simulink model "generic_src"  (Simulink 10.3)
settings: Solver=ode45  StartTime=0.0  StopTime=inf  RelTol=1e-3  EnableMultiTasking=on
undefined symbols (not defined in the file or in its folder): Area_Front, Area_Rear, ay_max_off, ay_max_on, ay_per_mu_max_off, ay_per_mu_max_on, Brake_ratio, brake_valve_ctrl_kP, cat1mode1_higher, cat1mode1_lower, cat1mode2_higher, cat1mode2_lower, cat1mode3_higher, cat1mode3_lower, cat2mode1_higher, cat2mode1_lower, cat2mode2_higher, cat2mode2_lower, cat2mode3_higher, cat2mode3_lower, delta_vel, diff_lock_fac, diff_lock_off, diff_lock_on, ESP_ctrl_kD, ESP_ctrl_kI, ESP_ctrl_kP, ESP_ctrl_restore_kI, ESP_min_throttle_fac, f_ax, f_slip, g, higherlimit_highvel, higherlimit_lowvel, highervel_fac, highervelocity_fac, InitialConditionForIntegrator, limit_acc, limit_selectlow, limit_starting, limit_vdiff, locktime_throttle, lowerlimit_highvel, lowerlimit_lowvel, lowervel_fac, lowervelocity_fac, min_throttle, MPS2KMPH, MSR_ctrl_kD, MSR_ctrl_kI, MSR_ctrl_kP, MSR_min_throttle_fac, PID_kP_sideslip, PID_kP_yawrate, RADpS2RpM, rBrake, RpM2RADpS, SH_SL_switch, sideslip_vel_corr, sidesplip_deviation_max ... (+35)
libraries: CarMaker4SL x136, simulink x55, simulink_extras x6
(part 2 of 9)

== system generic_src/CarMaker/IPG Vehicle/Brake/HydBrakeCU Example/CreateBus HydBrakeCU ==
  In : Inport
  BusCreator : BusCreator  Inputs=40
  Demux : Demux  Outputs=40
      settings: DisplayOption=none
  Ground{,1..5,7..12} (12 alike) : Ground
  Terminator{1..11,15} (12 alike) : Terminator
  Out : Outport  VectorParamsAs1DForOutWhenUnconnected=off
  wires:
  In/1 -> Demux/1
  BusCreator/1 -> Out/1
  Demux/1 -> BusCreator/1  "HydBrakeCU_Out Pedal"
  Demux/2 -> BusCreator/2  "HydBrakeCU_Out Park"
  Demux/3 -> BusCreator/3  "HydBrakeCU_Out Trq_BrakeReg_trg_FL"
  Demux/4 -> BusCreator/4  "HydBrakeCU_Out Trq_BrakeReg_trg_FR"
  Demux/5 -> BusCreator/5  "HydBrakeCU_Out Trq_BrakeReg_trg_RL"
  Demux/6 -> BusCreator/6  "HydBrakeCU_Out Trq_BrakeReg_trg_RR"
  Demux/7 -> BusCreator/7  "HydBrakeCU_Out Trq_DriveSrc_trg_d0"
  Demux/8 -> BusCreator/8  "HydBrakeCU_Out Trq_DriveSrc_trg_d1"
  Demux/9 -> BusCreator/9  "HydBrakeCU_Out Trq_DriveSrc_trg_d2"
  Demux/10 -> BusCreator/10  "HydBrakeCU_Out Trq_DriveSrc_trg_d3"
  Demux/11 -> BusCreator/11  "HydBrakeCU_Out Valve_FL_Inlet"
  Demux/12 -> BusCreator/12  "HydBrakeCU_Out Valve_FR_Inlet"
  Demux/13 -> BusCreator/13  "HydBrakeCU_Out Valve_RL_Inlet"
  Demux/14 -> BusCreator/14  "HydBrakeCU_Out Valve_RR_Inlet"
  Demux/15 -> BusCreator/15  "HydBrakeCU_Out Valve_FL_Outlet"
  Demux/16 -> BusCreator/16  "HydBrakeCU_Out Valve_FR_Outlet"
  Demux/17 -> BusCreator/17  "HydBrakeCU_Out Valve_RL_Outlet"
  Demux/18 -> BusCreator/18  "HydBrakeCU_Out Valve_RR_Outlet"
  Demux/19 -> BusCreator/19  "HydBrakeCU_Out Valve_PV_1"
  Demux/20 -> BusCreator/20  "HydBrakeCU_Out Valve_PV_2"
  Demux/21 -> BusCreator/21  "HydBrakeCU_Out Valve_SV_1"
  Demux/22 -> BusCreator/22  "HydBrakeCU_Out Valve_SV_2"
  Demux/23 -> BusCreator/23  "HydBrakeCU_Out Valve_V_1"
  Demux/24 -> BusCreator/24  "HydBrakeCU_Out Valve_V_2"
  Demux/25 -> BusCreator/25  "HydBrakeCU_Out Valve_V_3"
  Demux/26 -> BusCreator/26  "HydBrakeCU_Out Valve_V_4"
  Demux/27 -> BusCreator/27  "HydBrakeCU_Out PumpCtrl"
  Demux/28 -> BusCreator/28  "HydBrakeCU_Out BooSignal"
  Demux/40 -> Terminator6/1
  Demux/39 -> Terminator7/1
  Demux/38 -> Terminator8/1
  Demux/37 -> Terminator9/1
  Demux/36 -> Terminator10/1
  Demux/35 -> Terminator11/1
  Demux/31 -> Terminator15/1
  Demux/29 -> Terminator1/1
  Ground/1 -> BusCreator/29
  Ground1/1 -> BusCreator/30
  Ground2/1 -> BusCreator/31
  Ground3/1 -> BusCreator/32
  Ground4/1 -> BusCreator/33
  Ground5/1 -> BusCreator/34
  Ground12/1 -> BusCreator/35
  Ground7/1 -> BusCreator/36
  Ground8/1 -> BusCreator/37
  Ground9/1 -> BusCreator/38
  Ground10/1 -> BusCreator/39
  Ground11/1 -> BusCreator/40
  Demux/30 -> Terminator5/1
  Demux/32 -> Terminator2/1
  Demux/33 -> Terminator3/1
  Demux/34 -> Terminator4/1

== system generic_src/CarMaker/IPG Vehicle/Brake/HydBrakeCU Example/ESP Controller ==
  note: Quantities needed by this model, but not yet available
      | at program start on CM/HIL-ds100x. Define a dummy here,
      | they will be redefined later by CarMaker.
  HydBrakeCtrl_In : Inport
  Enable : EnablePort  StatesWhenEnabling=reset
  Define CM Dict1 : CarMaker4SL/Define CM Dict  xname=PT.Engine.Trq  xunit=Nm  xmono=off  xtype=Double4  xdvaplace=None  xnstates=0  xfirststate=0  xinitial=0
  Define CM Dict11 : CarMaker4SL/Define CM Dict  xname=PT.ECU.Load_lim_max  xmono=off  xtype=Double4  xdvaplace=PTC  xnstates=0  xfirststate=0  xinitial=0
  Define CM Dict2 : CarMaker4SL/Define CM Dict  xname=PT.Gen.DL.FDiff.DVA.Trq_A2B  xunit=Nm  xmono=off  xtype=Double4  xdvaplace=VC  xnstates=0  xfirststate=0  xinitial=0
  Define CM Dict3 : CarMaker4SL/Define CM Dict  xname=PT.Clutch.0.rotv_out  xunit=rad/s  xmono=off  xtype=Double4  xdvaplace=None  xnstates=0  xfirststate=0  xinitial=0
  ESP General System : Subsystem
  ESP Input Signals : Subsystem
  Ideal Input Signals : Subsystem
  Output Signals ESP : Subsystem
  User Input Signals1 : Subsystem
  Vehicle Input Parameter : Subsystem
  HydBrakeCU_Out : Outport  VectorParamsAs1DForOutWhenUnconnected=off
  wires:
  ESP Input Signals/1(ESP Signals) -> ESP General System/1(ESP Input Signals)
  User Input Signals1/1(User_In) -> ESP General System/2(User Input Signals)
  Vehicle Input Parameter/1(Vehicle Param) -> ESP General System/3(Vehicle Input Params)
  Ideal Input Signals/1(Ideal_In) -> ESP General System/4(Ideal_In)
  Output Signals ESP/1(HydBrakeCU_Out) -> HydBrakeCU_Out/1
  HydBrakeCtrl_In/1 -> ESP Input Signals/1(HydBrakeCtrl_In)
  ESP General System/1(ESP Out) -> Output Signals ESP/1(ESP Out)

== system generic_src/CarMaker/IPG Vehicle/Brake/HydBrakeCU Example/HydBrakeCtrl_In ==
  Sync_In : Inport
  CreateBus HydBrakeCU : Subsystem
  CreateBus HydBrakeCU_Cfg : Subsystem
  CreateBus HydBrakeCtrl_In : BusCreator  Inputs=2
  S-Function : S-Function  FunctionName=cm_hydbrakectrl_in  SFunctionDeploymentMode=off  EnableBusSupport=off
  HydBrakeCtrl_In : Outport  VectorParamsAs1DForOutWhenUnconnected=off
  wires:
  Sync_In/1 -> S-Function/1
  CreateBus HydBrakeCtrl_In/1 -> HydBrakeCtrl_In/1
  S-Function/1 -> CreateBus HydBrakeCU_Cfg/1(In)
  CreateBus HydBrakeCU_Cfg/1(Out) -> CreateBus HydBrakeCtrl_In/1  "HydBrakeCU_Cfg"
  S-Function/2 -> CreateBus HydBrakeCU/1(In)
  CreateBus HydBrakeCU/1(Out) -> CreateBus HydBrakeCtrl_In/2  "HydBrakeCU"

== system generic_src/CarMaker/IPG Vehicle/Brake/HydBrakeCU Example/HydBrakeCtrl_Out ==
  HydBrakeCU : Inport
  S-Function : S-Function  FunctionName=cm_hydbrakectrl_out  SFunctionDeploymentMode=off  EnableBusSupport=off
  wires:
  HydBrakeCU/1 -> S-Function/1

== system generic_src/CarMaker/IPG Vehicle/CarAndTrailer/CarAndTrailerUpd/CreateBus Brake.IF.In ==
  In : Inport
  BusCreator : BusCreator  Inputs=9
  Demux : Demux  Outputs=9
      settings: DisplayOption=none
  Out : Outport  VectorParamsAs1DForOutWhenUnconnected=off
  wires:
  Demux/9 -> BusCreator/9  "Brake IF Trq_Reg RR"
  Demux/8 -> BusCreator/8  "Brake IF Trq_Reg RL"
  Demux/7 -> BusCreator/7  "Brake IF Trq_Reg FR"
  Demux/6 -> BusCreator/6  "Brake IF Trq_Reg FL"
  Demux/5 -> BusCreator/5  "Brake IF Trq_Reg_max RR"
  Demux/4 -> BusCreator/4  "Brake IF Trq_Reg_max RL"
  Demux/3 -> BusCreator/3  "Brake IF Trq_Reg_max FR"
  Demux/2 -> BusCreator/2  "Brake IF Trq_Reg_max FL"
  Demux/1 -> BusCreator/1  "Brake IF T_env"
  BusCreator/1 -> Out/1
  In/1 -> Demux/1

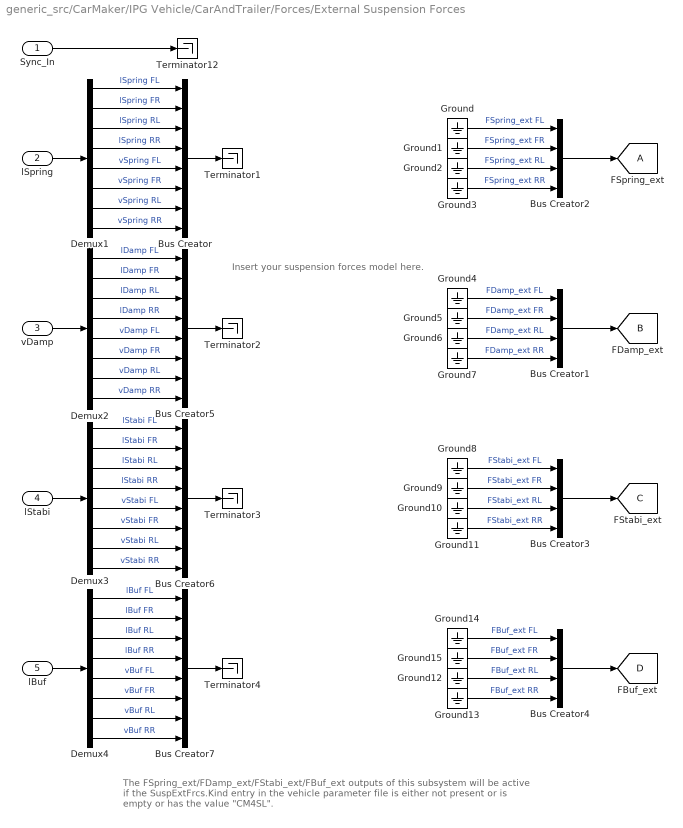
== system generic_src/CarMaker/IPG Vehicle/CarAndTrailer/Forces/External Suspension Forces ==
  note: The FSpring_ext/FDamp_ext/FStabi_ext/FBuf_ext outputs of this subsystem will be
      | active if the SuspExtFrcs.Kind entry in the vehicle parameter file
      | is either not present or is empty or has the value "CM4SL".
  note: Insert your suspension forces model here.
  Sync_In : Inport
  lSpring : Inport  Port=2
  vDamp : Inport  Port=3
  lStabi : Inport  Port=4
  lBuf : Inport  Port=5
  Bus Creator{,5..7} (4 alike) : BusCreator  Inputs=8
  Bus Creator{1..4} (4 alike) : BusCreator  Inputs=4
  Demux{1..4} (4 alike) : Demux  Outputs=8
      settings: DisplayOption=none
  Ground{,1..15} (16 alike) : Ground
  Terminator{1..4,12} (5 alike) : Terminator
  tag scope: A=global, B=global, C=global, D=global
  wires:
  Bus Creator7/1 -> Terminator4/1
  Bus Creator6/1 -> Terminator3/1
  Bus Creator5/1 -> Terminator2/1
  Bus Creator/1 -> Terminator1/1
  Demux4/8 -> Bus Creator7/8  "vBuf RR"
  Demux4/7 -> Bus Creator7/7  "vBuf RL"
  Demux4/6 -> Bus Creator7/6  "vBuf FR"
  Demux4/5 -> Bus Creator7/5  "vBuf FL"
  Demux3/8 -> Bus Creator6/8  "vStabi RR"
  Demux3/7 -> Bus Creator6/7  "vStabi RL"
  Demux3/6 -> Bus Creator6/6  "vStabi FR"
  Demux3/5 -> Bus Creator6/5  "vStabi FL"
  Demux2/8 -> Bus Creator5/8  "vDamp RR"
  Demux2/7 -> Bus Creator5/7  "vDamp RL"
  Demux2/6 -> Bus Creator5/6  "vDamp FR"
  Demux2/5 -> Bus Creator5/5  "vDamp FL"
  Demux1/8 -> Bus Creator/8  "vSpring RR"
  Demux1/7 -> Bus Creator/7  "vSpring RL"
  Demux1/6 -> Bus Creator/6  "vSpring FR"
  Demux1/5 -> Bus Creator/5  "vSpring FL"
  Demux2/4 -> Bus Creator5/4  "lDamp RR"
  Demux2/3 -> Bus Creator5/3  "lDamp RL"
  Demux2/2 -> Bus Creator5/2  "lDamp FR"
  Demux2/1 -> Bus Creator5/1  "lDamp FL"
  Demux1/4 -> Bus Creator/4  "lSpring RR"
  Demux1/3 -> Bus Creator/3  "lSpring RL"
  Demux1/2 -> Bus Creator/2  "lSpring FR"
  Demux1/1 -> Bus Creator/1  "lSpring FL"
  Demux3/4 -> Bus Creator6/4  "lStabi RR"
  Demux3/3 -> Bus Creator6/3  "lStabi RL"
  Demux3/2 -> Bus Creator6/2  "lStabi FR"
  Demux3/1 -> Bus Creator6/1  "lStabi FL"
  lStabi/1 -> Demux3/1
  vDamp/1 -> Demux2/1
  lSpring/1 -> Demux1/1
  Demux4/4 -> Bus Creator7/4  "lBuf RR"
  Demux4/3 -> Bus Creator7/3  "lBuf RL"
  Demux4/2 -> Bus Creator7/2  "lBuf FR"
  Demux4/1 -> Bus Creator7/1  "lBuf FL"
  lBuf/1 -> Demux4/1
  Ground14/1 -> Bus Creator4/1  "FBuf_ext FL"
  Ground15/1 -> Bus Creator4/2  "FBuf_ext FR"
  Ground12/1 -> Bus Creator4/3  "FBuf_ext RL"
  Ground13/1 -> Bus Creator4/4  "FBuf_ext RR"
  Bus Creator4/1 -> [D]
  Sync_In/1 -> Terminator12/1
  Bus Creator2/1 -> [A]
  Ground/1 -> Bus Creator2/1  "FSpring_ext FL"
  Ground1/1 -> Bus Creator2/2  "FSpring_ext FR"
  Ground2/1 -> Bus Creator2/3  "FSpring_ext RL"
  Ground3/1 -> Bus Creator2/4  "FSpring_ext RR"
  Ground4/1 -> Bus Creator1/1  "FDamp_ext FL"
  Ground5/1 -> Bus Creator1/2  "FDamp_ext FR"
  Ground6/1 -> Bus Creator1/3  "FDamp_ext RL"
  Ground7/1 -> Bus Creator1/4  "FDamp_ext RR"
  Bus Creator1/1 -> [B]
  Ground8/1 -> Bus Creator3/1  "FStabi_ext FL"
  Ground9/1 -> Bus Creator3/2  "FStabi_ext FR"
  Ground10/1 -> Bus Creator3/3  "FStabi_ext RL"
  Ground11/1 -> Bus Creator3/4  "FStabi_ext RR"
  Bus Creator3/1 -> [C]

== system generic_src/CarMaker/IPG Vehicle/CarAndTrailer/Forces/Suspension Forces ==
  note: <Your model here>
  note: <Your model here>
  Sync_In : Inport
  Bus Creator{,1..3,9..10} (6 alike) : BusCreator  Inputs=4
  Bus Creator{4..7} (4 alike) : BusCreator  Inputs=6
  Demux{,1..5} (6 alike) : Demux
  Demux{6..9} (4 alike) : Demux  Outputs=6
  Suspension Control Unit : S-Function  FunctionName=CM_Sfun  Parameters='ForcesSuspControl'  SFunctionDeploymentMode=off  EnableBusSupport=off
  Suspension External Forces Update : Subsystem
  Suspension Force Elements : S-Function  FunctionName=CM_Sfun  Parameters='ForcesSusp'  SFunctionDeploymentMode=off  EnableBusSupport=off
  Suspension Force Elements Update : S-Function  FunctionName=CM_Sfun  Parameters='ForcesSuspUpd'  SFunctionDeploymentMode=off  EnableBusSupport=off
  Sync_Out : Outport  VectorParamsAs1DForOutWhenUnconnected=off
  wires:
  Demux9/2 -> Bus Creator7/2  "RR DamperForce"
  Suspension Force Elements/4 -> ?
  Suspension External Forces Update/1(Out1) -> Suspension Force Elements Update/3
  Demux9/5 -> Bus Creator7/5  "RR ParasiticStiffForce"
  ? -> Suspension Force Elements Update/5
  Demux4/2 -> Bus Creator2/2  "RL DamperCtrlOut"
  Demux6/2 -> Bus Creator4/2  "FL DamperForce"
  Demux3/1 -> Bus Creator1/1  "FR SpringCtrlOut"
  Demux7/1 -> Bus Creator5/1  "FR SpringForce"
  Demux/3 -> Demux4/1  "RL"
  Demux2/1 -> Bus Creator/1  "FL SpringCtrlOut"
  Bus Creator3/1 -> Bus Creator9/4
  Demux4/1 -> Bus Creator2/1  "RL SpringCtrlOut"
  Demux/2 -> Demux3/1  "FR"
  Demux6/6 -> Bus Creator4/6  "FL ParasiticFricForce"
  Demux1/4 -> Demux9/1  "RR"
  Demux6/3 -> Bus Creator4/3  "FL StabiForce"
  Suspension Control Unit/2 -> Demux/1
  Demux3/3 -> Bus Creator1/3  "FR StabiCtrlOut"
  Demux2/4 -> Bus Creator/4  "FL BufferCtrlOut"
  Demux8/3 -> Bus Creator6/3  "RL StabiForce"
  Demux7/5 -> Bus Creator5/5  "FR ParasiticStiffForce"
  Demux6/1 -> Bus Creator4/1  "FL SpringForce"
  Suspension Force Elements/1 -> Suspension Force Elements Update/1
  Suspension Control Unit/1 -> Suspension Force Elements/1
  Demux4/4 -> Bus Creator2/4  "RL BufferCtrlOut"
  Demux3/2 -> Bus Creator1/2  "FR DamperCtrlOut"
  Demux7/4 -> Bus Creator5/4  "FR BufferForce"
  Demux9/1 -> Bus Creator7/1  "RR SpringForce"
  Bus Creator2/1 -> Bus Creator9/3
  Demux8/2 -> Bus Creator6/2  "RL DamperForce"
  ? -> Suspension Force Elements/4
  Demux1/2 -> Demux7/1  "FR"
  Demux/1 -> Demux2/1  "FL"
  Demux5/1 -> Bus Creator3/1  "RR SpringCtrlOut"
  Bus Creator1/1 -> Bus Creator9/2
  Suspension Control Unit/4 -> ?
  Sync_In/1 -> Suspension Control Unit/1
  Demux7/3 -> Bus Creator5/3  "FR StabiForce"
  Bus Creator5/1 -> Bus Creator10/2
  Demux8/6 -> Bus Creator6/6  "RL ParasiticFricForce"
  Demux9/6 -> Bus Creator7/6  "RR ParasiticFricForce"
  Suspension Force Elements/3 -> ?
  Bus Creator10/1 -> Suspension Force Elements Update/2
  ? -> Suspension Force Elements Update/4
  Demux9/4 -> Bus Creator7/4  "RR BufferForce"
  Demux7/2 -> Bus Creator5/2  "FR DamperForce"
  Demux7/6 -> Bus Creator5/6  "FR ParasiticFricForce"
  Demux2/3 -> Bus Creator/3  "FL StabiCtrlOut"
  Demux5/2 -> Bus Creator3/2  "RR DamperCtrlOut"
  Demux6/4 -> Bus Creator4/4  "FL BufferForce"
  Demux5/3 -> Bus Creator3/3  "RR StabiCtrlOut"
  Bus Creator4/1 -> Bus Creator10/1
  Suspension Force Elements/2 -> Demux1/1
  ? -> Suspension Force Elements/3
  Demux9/3 -> Bus Creator7/3  "RR StabiForce"
  Suspension Control Unit/3 -> ?
  Demux8/4 -> Bus Creator6/4  "RL BufferForce"
  Suspension Force Elements Update/1 -> Sync_Out/1
  Demux6/5 -> Bus Creator4/5  "FL ParasiticStiffForce"
  Demux5/4 -> Bus Creator3/4  "RR BufferCtrlOut"
  Demux4/3 -> Bus Creator2/3  "RL StabiCtrlOut"
  Bus Creator6/1 -> Bus Creator10/3
  Demux3/4 -> Bus Creator1/4  "FR BufferCtrlOut"
  Demux2/2 -> Bus Creator/2  "FL DamperCtrlOut"
  Bus Creator9/1 -> Suspension Force Elements/2
  Bus Creator/1 -> Bus Creator9/1
  Demux8/5 -> Bus Creator6/5  "RL ParasiticStiffForce"
  Demux1/1 -> Demux6/1  "FL"
  Demux1/3 -> Demux8/1  "RL"
  Demux8/1 -> Bus Creator6/1  "RL SpringForce"
  Demux/4 -> Demux5/1  "RR"
  Bus Creator7/1 -> Bus Creator10/4

== system generic_src/CarMaker/IPG Vehicle/CarAndTrailer/Forces/Tires ==
  note: The TireXX_Out signals will only be used if FileIdent is "CarMaker-Tire-CM4SL" in the tire parameter file!
      | An example parameter file can be found in Data/Tire/DT_CM4SL_UserTire.
  Sync_In : Inport
  TireFL_In : Inport  Port=2
  TireFR_In : Inport  Port=3
  TireRL_In : Inport  Port=4
  TireRR_In : Inport  Port=5
  Bus Creator{1..4} (4 alike) : BusCreator  Inputs=11
  Demux{1..3,8} (4 alike) : Demux  Outputs=7
      settings: DisplayOption=none
  TireFL : Subsystem
  TireFR : Subsystem
  TireRL : Subsystem
  TireRR : Subsystem
  TireFL_Out : Outport  VectorParamsAs1DForOutWhenUnconnected=off
  TireFR_Out : Outport  Port=2  VectorParamsAs1DForOutWhenUnconnected=off
  TireRL_Out : Outport  Port=3  VectorParamsAs1DForOutWhenUnconnected=off
  TireRR_Out : Outport  Port=4  VectorParamsAs1DForOutWhenUnconnected=off
  wires:
  Sync_In/1 -> TireRR/1(Sync_In), TireRL/1(Sync_In), TireFR/1(Sync_In), TireFL/1(Sync_In)
  Bus Creator4/1 -> TireRR_Out/1
  Bus Creator2/1 -> TireRL_Out/1
  Bus Creator1/1 -> TireFR_Out/1
  Demux3/5 -> TireRR/6(Rim_turnv)  "Tire_In Rim_turnv"
  Demux3/4 -> TireRR/5(Rim_rotv)  "Tire_In Rim_rotv"
  Demux3/1 -> TireRR/2(Load)  "Tire_In Load"
  Demux3/7 -> TireRR/8(muRoad)  "Tire_In mu"
  Demux3/6 -> TireRR/7(InclinAngle)  "Tire_In Camber"
  Demux3/2 -> TireRR/3(vxtrans)  "Tire_In vxtrans"
  Demux3/3 -> TireRR/4(vytrans)  "Tire_In vytrans"
  TireRR/11(AlignTrq) -> Bus Creator4/11  "Tire_Out AlignTrq"
  TireRR/10(RollResist) -> Bus Creator4/10  "Tire_Out RollResist"
  TireRR/9(OverturnTrq) -> Bus Creator4/9  "Tire_Out OverturnTrq"
  TireRR/8(LoadFrc) -> Bus Creator4/8  "Tire_Out LoadFrc"
  TireRR/7(SideFrc) -> Bus Creator4/7  "Tire_Out SideFrc"
  TireRR/6(LongFrc) -> Bus Creator4/6  "Tire_Out LongFrc"
  TireRR/5(vBelt) -> Bus Creator4/5  "Tire_Out vBelt"
  TireRR/4(rBelt_eff) -> Bus Creator4/4  "Tire_Out rBelt_eff"
  TireRR/3(TurnSlp) -> Bus Creator4/3  "Tire_Out TurnSlp"
  TireRR/1(Slp) -> Bus Creator4/1  "Tire_Out Slp"
  TireRR/2(Alpha) -> Bus Creator4/2  "Tire_Out Alpha"
  Demux2/5 -> TireRL/6(Rim_turnv)  "Tire_In Rim_turnv"
  Demux2/4 -> TireRL/5(Rim_rotv)  "Tire_In Rim_rotv"
  Demux2/1 -> TireRL/2(Load)  "Tire_In Load"
  Demux2/7 -> TireRL/8(muRoad)  "Tire_In mu"
  Demux2/6 -> TireRL/7(InclinAngle)  "Tire_In Camber"
  Demux2/2 -> TireRL/3(vxtrans)  "Tire_In vxtrans"
  Demux2/3 -> TireRL/4(vytrans)  "Tire_In vytrans"
  TireRL/11(AlignTrq) -> Bus Creator2/11  "Tire_Out AlignTrq"
  TireRL/10(RollResist) -> Bus Creator2/10  "Tire_Out RollResist"
  TireRL/9(OverturnTrq) -> Bus Creator2/9  "Tire_Out OverturnTrq"
  TireRL/8(LoadFrc) -> Bus Creator2/8  "Tire_Out LoadFrc"
  TireRL/7(SideFrc) -> Bus Creator2/7  "Tire_Out SideFrc"
  TireRL/6(LongFrc) -> Bus Creator2/6  "Tire_Out LongFrc"
  TireRL/5(vBelt) -> Bus Creator2/5  "Tire_Out vBelt"
  TireRL/4(rBelt_eff) -> Bus Creator2/4  "Tire_Out rBelt_eff"
  TireRL/3(TurnSlp) -> Bus Creator2/3  "Tire_Out TurnSlp"
  TireRL/1(Slp) -> Bus Creator2/1  "Tire_Out Slp"
  TireRL/2(Alpha) -> Bus Creator2/2  "Tire_Out Alpha"
  Demux1/5 -> TireFR/6(Rim_turnv)  "Tire_In Rim_turnv"
  Demux1/4 -> TireFR/5(Rim_rotv)  "Tire_In Rim_rotv"
  Demux1/1 -> TireFR/2(Load)  "Tire_In Load"
  Demux1/7 -> TireFR/8(muRoad)  "Tire_In mu"
  Demux1/6 -> TireFR/7(InclinAngle)  "Tire_In Camber"
  Demux1/2 -> TireFR/3(vxtrans)  "Tire_In vxtrans"
  Demux1/3 -> TireFR/4(vytrans)  "Tire_In vytrans"
  TireFR/11(AlignTrq) -> Bus Creator1/11  "Tire_Out AlignTrq"
  TireFR/10(RollResist) -> Bus Creator1/10  "Tire_Out RollResist"
  TireFR/9(OverturnTrq) -> Bus Creator1/9  "Tire_Out OverturnTrq"
  TireFR/8(LoadFrc) -> Bus Creator1/8  "Tire_Out LoadFrc"
  TireFR/7(SideFrc) -> Bus Creator1/7  "Tire_Out SideFrc"
  TireFR/6(LongFrc) -> Bus Creator1/6  "Tire_Out LongFrc"
  TireFR/5(vBelt) -> Bus Creator1/5  "Tire_Out vBelt"
  TireFR/4(rBelt_eff) -> Bus Creator1/4  "Tire_Out rBelt_eff"
  TireFR/3(TurnSlp) -> Bus Creator1/3  "Tire_Out TurnSlp"
  TireFR/1(Slp) -> Bus Creator1/1  "Tire_Out Slp"
  TireFR/2(Alpha) -> Bus Creator1/2  "Tire_Out Alpha"
  Demux8/5 -> TireFL/6(Rim_turnv)  "Tire_In Rim_turnv"
  Demux8/4 -> TireFL/5(Rim_rotv)  "Tire_In Rim_rotv"
  TireFL_In/1 -> Demux8/1
  Demux8/1 -> TireFL/2(Load)  "Tire_In Load"
  Demux8/7 -> TireFL/8(muRoad)  "Tire_In mu"
  Demux8/6 -> TireFL/7(InclinAngle)  "Tire_In Camber"
  Demux8/2 -> TireFL/3(vxtrans)  "Tire_In vxtrans"
  Demux8/3 -> TireFL/4(vytrans)  "Tire_In vytrans"
  TireFL/11(AlignTrq) -> Bus Creator3/11  "Tire_Out AlignTrq"
  TireFL/10(RollResist) -> Bus Creator3/10  "Tire_Out RollResist"
  TireFL/9(OverturnTrq) -> Bus Creator3/9  "Tire_Out OverturnTrq"
  TireFL/8(LoadFrc) -> Bus Creator3/8  "Tire_Out LoadFrc"
  TireFL/7(SideFrc) -> Bus Creator3/7  "Tire_Out SideFrc"
  TireFL/6(LongFrc) -> Bus Creator3/6  "Tire_Out LongFrc"
  TireFL/5(vBelt) -> Bus Creator3/5  "Tire_Out vBelt"
  TireFL/4(rBelt_eff) -> Bus Creator3/4  "Tire_Out rBelt_eff"
  TireFL/3(TurnSlp) -> Bus Creator3/3  "Tire_Out TurnSlp"
  TireFL/1(Slp) -> Bus Creator3/1  "Tire_Out Slp"
  TireFL/2(Alpha) -> Bus Creator3/2  "Tire_Out Alpha"
  Bus Creator3/1 -> TireFL_Out/1
  TireFR_In/1 -> Demux1/1
  TireRL_In/1 -> Demux2/1
  TireRR_In/1 -> Demux3/1

== system generic_src/CarMaker/IPG Vehicle/CarAndTrailer/Forces/Vehicle Forces ==
  Sync_In : Inport
  Bus Creator1 : BusCreator  Inputs=12
  Bus Creator8 : BusCreator  Inputs=16
  BusCreator1 : BusCreator  Inputs=4
  BusCreator2 : BusCreator  Inputs=9
  Demux : Demux  Outputs=16
      settings: DisplayOption=none
  Demux1 : Demux  Outputs=12
      settings: DisplayOption=none
  Demux2 : Demux  Outputs=13
      settings: DisplayOption=none
  Forces : S-Function  FunctionName=CM_Sfun  Parameters='Forces'  SFunctionDeploymentMode=off  EnableBusSupport=off
  Terminator : Terminator
  Sync_Out : Outport  VectorParamsAs1DForOutWhenUnconnected=off
  Car.Virtual : Outport  Port=2  VectorParamsAs1DForOutWhenUnconnected=off
  Car.Aero : Outport  Port=3  VectorParamsAs1DForOutWhenUnconnected=off
  Car.Load : Outport  Port=4  VectorParamsAs1DForOutWhenUnconnected=off
  wires:
  BusCreator1/1 -> Terminator/1  "Aero IF (in)"
  Demux2/13 -> BusCreator2/9  "car Aero Trq_1 z"
  Demux2/12 -> BusCreator2/8  "car Aero Trq_1 y"
  Demux2/11 -> BusCreator2/7  "car Aero Trq_1 x"
  Demux2/10 -> BusCreator2/6  "car Aero Frc_1 z"
  Demux2/9 -> BusCreator2/5  "car Aero Frc_1 y"
  Demux2/8 -> BusCreator2/4  "car Aero Frc_1 x"
  Demux2/7 -> BusCreator2/3  "car Aero PoA_1 z"
  Demux2/6 -> BusCreator2/2  "car Aero PoA_1 y"
  Demux2/5 -> BusCreator2/1  "car Aero PoA_1 x"
  Demux2/4 -> BusCreator1/4  "car Aero tau_1"
  Demux2/3 -> BusCreator1/3  "car Aero ApproachVel_1 z"
  Demux2/2 -> BusCreator1/2  "car Aero ApproachVel_1 y"
  Demux2/1 -> BusCreator1/1  "car Aero ApproachVel_1 x"
  Demux/16 -> Bus Creator8/16  "Car Load_3 tz"
  Demux/15 -> Bus Creator8/15  "Car Load_3 ty"
  Demux/14 -> Bus Creator8/14  "Car Load_3 tx"
  Demux/13 -> Bus Creator8/13  "Car Load_3 mass"
  Demux1/12 -> Bus Creator1/12  "Car Virtual Trq_0 z"
  Demux1/11 -> Bus Creator1/11  "Car Virtual Trq_0 y"
  Demux1/10 -> Bus Creator1/10  "Car Virtual Trq_0 x"
  Demux1/9 -> Bus Creator1/9  "Car Virtual Trq_1 z"
  Demux1/8 -> Bus Creator1/8  "Car Virtual Trq_1 y"
  Demux1/7 -> Bus Creator1/7  "Car Virtual Trq_1 x"
  Demux1/6 -> Bus Creator1/6  "Car Virtual Frc_0 z"
  Demux1/5 -> Bus Creator1/5  "Car Virtual Frc_0 y"
  Demux1/4 -> Bus Creator1/4  "Car Virtual Frc_0 x"
  Sync_In/1 -> Forces/1
  Forces/1 -> Sync_Out/1
  BusCreator2/1 -> Car.Aero/1
  Demux1/1 -> Bus Creator1/1  "Car Virtual Frc_1 x"
  Demux1/2 -> Bus Creator1/2  "Car Virtual Frc_1 y"
  Demux1/3 -> Bus Creator1/3  "Car Virtual Frc_1 z"
  Forces/3 -> Demux2/1
  Forces/2 -> Demux1/1
  Bus Creator1/1 -> Car.Virtual/1
  Bus Creator8/1 -> Car.Load/1
  Demux/1 -> Bus Creator8/1  "Car Load_0 mass"
  Demux/2 -> Bus Creator8/2  "Car Load_0 tx"
  Demux/3 -> Bus Creator8/3  "Car Load_0 ty"
  Demux/4 -> Bus Creator8/4  "Car Load_0 tz"
  Demux/5 -> Bus Creator8/5  "Car Load_1 mass"
  Demux/6 -> Bus Creator8/6  "Car Load_1 tx"
  Demux/7 -> Bus Creator8/7  "Car Load_1 ty"
  Demux/8 -> Bus Creator8/8  "Car Load_1 tz"
  Demux/9 -> Bus Creator8/9  "Car Load_2 mass"
  Demux/10 -> Bus Creator8/10  "Car Load_2 tx"
  Demux/11 -> Bus Creator8/11  "Car Load_2 ty"
  Demux/12 -> Bus Creator8/12  "Car Load_2 tz"
  Forces/4 -> Demux/1

== system generic_src/CarMaker/IPG Vehicle/CarAndTrailer/Trailer/CreateBus Car.Hitch.FrcTrq ==
  In1 : Inport
  Bus Creator7 : BusCreator  Inputs=6
  Demux7 : Demux  Outputs=6
      settings: DisplayOption=none
  Out1 : Outport  VectorParamsAs1DForOutWhenUnconnected=off
  wires:
  In1/1 -> Demux7/1
  Bus Creator7/1 -> Out1/1
  Demux7/6 -> Bus Creator7/6  "Car Hitch Trq2Car z"
  Demux7/5 -> Bus Creator7/5  "Car Hitch Trq2Car y"
  Demux7/4 -> Bus Creator7/4  "Car Hitch Trq2Car x"
  Demux7/3 -> Bus Creator7/3  "Car Hitch Frc2Car z"
  Demux7/2 -> Bus Creator7/2  "Car Hitch Frc2Car y"
  Demux7/1 -> Bus Creator7/1  "Car Hitch Frc2Car x"

== system generic_src/CarMaker/IPG Vehicle/CarAndTrailer/Trailer/CreateBus Vhcl.Motion ==
  In1 : Inport
  BusCreator : BusCreator  Inputs=15
  Demux : Demux  Outputs=15
      settings: DisplayOption=none
  Out1 : Outport  VectorParamsAs1DForOutWhenUnconnected=off
  wires:
  Demux/15 -> BusCreator/15  "Vhcl YawAcc"
  Demux/14 -> BusCreator/14  "Vhcl YawVel"
  Demux/13 -> BusCreator/13  "Vhcl Yaw"
  Demux/12 -> BusCreator/12  "Vhcl PitchAcc"
  Demux/11 -> BusCreator/11  "Vhcl PitchVel"
  Demux/10 -> BusCreator/10  "Vhcl Pitch"
  Demux/9 -> BusCreator/9  "Vhcl RollAcc"
  Demux/8 -> BusCreator/8  "Vhcl RollVel"
  Demux/7 -> BusCreator/7  "Vhcl Roll"
  Demux/6 -> BusCreator/6  "Vhcl Hitch_Pos z"
  Demux/5 -> BusCreator/5  "Vhcl Hitch_Pos y"
  Demux/4 -> BusCreator/4  "Vhcl Hitch_Pos x"
  Demux/3 -> BusCreator/3  "Vhcl sRoad"
  Demux/2 -> BusCreator/2  "Vhcl Distance"
  Demux/1 -> BusCreator/1  "Vhcl v"
  In1/1 -> Demux/1
  BusCreator/1 -> Out1/1

== system generic_src/CarMaker/IPG Vehicle/CarAndTrailer/Trailer/CreateBus Vhcl.PoI ==
  In1 : Inport
  Bus Creator3 : BusCreator  Inputs=18
  Demux3 : Demux  Outputs=18
      settings: DisplayOption=none
  Out1 : Outport  VectorParamsAs1DForOutWhenUnconnected=off
  wires:
  Demux3/18 -> Bus Creator3/18  "Vhcl PoI_GCS Elev"
  Demux3/17 -> Bus Creator3/17  "Vhcl PoI_GCS Lat"
  Demux3/16 -> Bus Creator3/16  "Vhcl PoI_GCS Long"
  Demux3/15 -> Bus Creator3/15  "Vhcl PoI_Acc_1 z"
  Demux3/14 -> Bus Creator3/14  "Vhcl PoI_Acc_1 y"
  Demux3/13 -> Bus Creator3/13  "Vhcl PoI_Acc_1 x"
  Demux3/12 -> Bus Creator3/12  "Vhcl PoI_Vel_1 z"
  Demux3/11 -> Bus Creator3/11  "Vhcl PoI_Vel_1 y"
  Demux3/10 -> Bus Creator3/10  "Vhcl PoI_Vel_1 x"
  Demux3/9 -> Bus Creator3/9  "Vhcl PoI_Acc z"
  Demux3/8 -> Bus Creator3/8  "Vhcl PoI_Acc y"
  Demux3/7 -> Bus Creator3/7  "Vhcl PoI_Acc x"
  Demux3/6 -> Bus Creator3/6  "Vhcl PoI_Vel z"
  Demux3/5 -> Bus Creator3/5  "Vhcl PoI_Vel y"
  Demux3/4 -> Bus Creator3/4  "Vhcl PoI_Vel x"
  Demux3/3 -> Bus Creator3/3  "Vhcl PoI_Pos z"
  Demux3/2 -> Bus Creator3/2  "Vhcl PoI_Pos y"
  In1/1 -> Demux3/1
  Bus Creator3/1 -> Out1/1
  Demux3/1 -> Bus Creator3/1  "Vhcl PoI_Pos x"

== system generic_src/CarMaker/IPG Vehicle/CarAndTrailer/Trailer/CreateBus Vhcl.Steering ==
  In1 : Inport
  Bus Creator3 : BusCreator  Inputs=4
  Demux : Demux
      settings: DisplayOption=none
  Out1 : Outport  VectorParamsAs1DForOutWhenUnconnected=off
  wires:
  Bus Creator3/1 -> Out1/1
  Demux/1 -> Bus Creator3/1  "Vhcl Steering Ang"
  Demux/3 -> Bus Creator3/3  "Vhcl Steering AngAcc"
  Demux/2 -> Bus Creator3/2  "Vhcl Steering AngVel"
  Demux/4 -> Bus Creator3/4  "Vhcl Steering Trq"
  In1/1 -> Demux/1

== system generic_src/CarMaker/IPG Vehicle/CarAndTrailer/Trailer/CreateBus Vhcl.Wheel.FL ==
  In1 : Inport
  Bus Creator3 : BusCreator  Inputs=14
  Demux3 : Demux  Outputs=14
      settings: DisplayOption=none
  Out1 : Outport  VectorParamsAs1DForOutWhenUnconnected=off
  wires:
  Demux3/14 -> Bus Creator3/14  "Vhcl Wheel FL Trq_WhlBearing"
  Demux3/13 -> Bus Creator3/13  "Vhcl Wheel FL Trq_T2W"
  Demux3/12 -> Bus Creator3/12  "Vhcl Wheel FL SideSlip"
  Demux3/11 -> Bus Creator3/11  "Vhcl Wheel FL LongSlip"
  Demux3/10 -> Bus Creator3/10  "Vhcl Wheel FL vBelt"
  Demux3/9 -> Bus Creator3/9  "Vhcl Wheel FL Fz"
  Demux3/8 -> Bus Creator3/8  "Vhcl Wheel FL Fy"
  Demux3/7 -> Bus Creator3/7  "Vhcl Wheel FL Fx"
  Demux3/6 -> Bus Creator3/6  "Vhcl Wheel FL r_zxy z"
  Demux3/5 -> Bus Creator3/5  "Vhcl Wheel FL r_zxy y"
  Demux3/4 -> Bus Creator3/4  "Vhcl Wheel FL r_zxy x"
  Demux3/3 -> Bus Creator3/3  "Vhcl Wheel FL t z"
  Demux3/2 -> Bus Creator3/2  "Vhcl Wheel FL t y"
  In1/1 -> Demux3/1
  Bus Creator3/1 -> Out1/1
  Demux3/1 -> Bus Creator3/1  "Vhcl Wheel FL t x"

== system generic_src/CarMaker/IPG Vehicle/CarAndTrailer/Trailer/CreateBus Vhcl.Wheel.FR ==
  In1 : Inport
  Bus Creator3 : BusCreator  Inputs=14
  Demux3 : Demux  Outputs=14
      settings: DisplayOption=none
  Out1 : Outport  VectorParamsAs1DForOutWhenUnconnected=off
  wires:
  Demux3/14 -> Bus Creator3/14  "Vhcl Wheel FR Trq_WhlBearing"
  Demux3/13 -> Bus Creator3/13  "Vhcl Wheel FR Trq_T2W"
  Demux3/12 -> Bus Creator3/12  "Vhcl Wheel FR SideSlip"
  Demux3/11 -> Bus Creator3/11  "Vhcl Wheel FR LongSlip"
  Demux3/10 -> Bus Creator3/10  "Vhcl Wheel FR vBelt"
  Demux3/9 -> Bus Creator3/9  "Vhcl Wheel FR Fz"
  Demux3/8 -> Bus Creator3/8  "Vhcl Wheel FR Fy"
  Demux3/7 -> Bus Creator3/7  "Vhcl Wheel FR Fx"
  Demux3/6 -> Bus Creator3/6  "Vhcl Wheel FR r_zxy z"
  Demux3/5 -> Bus Creator3/5  "Vhcl Wheel FR r_zxy y"
  Demux3/4 -> Bus Creator3/4  "Vhcl Wheel FR r_zxy x"
  Demux3/3 -> Bus Creator3/3  "Vhcl Wheel FR t z"
  Demux3/2 -> Bus Creator3/2  "Vhcl Wheel FR t y"
  In1/1 -> Demux3/1
  Bus Creator3/1 -> Out1/1
  Demux3/1 -> Bus Creator3/1  "Vhcl Wheel FR t x"

== system generic_src/CarMaker/IPG Vehicle/CarAndTrailer/Trailer/CreateBus Vhcl.Wheel.RL ==
  In1 : Inport
  Bus Creator3 : BusCreator  Inputs=14
  Demux3 : Demux  Outputs=14
      settings: DisplayOption=none
  Out1 : Outport  VectorParamsAs1DForOutWhenUnconnected=off
  wires:
  Demux3/14 -> Bus Creator3/14  "Vhcl Wheel RL Trq_WhlBearing"
  Demux3/13 -> Bus Creator3/13  "Vhcl Wheel RL Trq_T2W"
  Demux3/12 -> Bus Creator3/12  "Vhcl Wheel RL SideSlip"
  Demux3/11 -> Bus Creator3/11  "Vhcl Wheel RL LongSlip"
  Demux3/10 -> Bus Creator3/10  "Vhcl Wheel RL vBelt"
  Demux3/9 -> Bus Creator3/9  "Vhcl Wheel RL Fz"
  Demux3/8 -> Bus Creator3/8  "Vhcl Wheel RL Fy"
  Demux3/7 -> Bus Creator3/7  "Vhcl Wheel RL Fx"
  Demux3/6 -> Bus Creator3/6  "Vhcl Wheel RL r_zxy z"
  Demux3/5 -> Bus Creator3/5  "Vhcl Wheel RL r_zxy y"
  Demux3/4 -> Bus Creator3/4  "Vhcl Wheel RL r_zxy x"
  Demux3/3 -> Bus Creator3/3  "Vhcl Wheel RL t z"
  Demux3/2 -> Bus Creator3/2  "Vhcl Wheel RL t y"
  In1/1 -> Demux3/1
  Bus Creator3/1 -> Out1/1
  Demux3/1 -> Bus Creator3/1  "Vhcl Wheel RL t x"

== system generic_src/CarMaker/IPG Vehicle/CarAndTrailer/Trailer/CreateBus Vhcl.Wheel.RR ==
  In1 : Inport
  Bus Creator3 : BusCreator  Inputs=14
  Demux3 : Demux  Outputs=14
      settings: DisplayOption=none
  Out1 : Outport  VectorParamsAs1DForOutWhenUnconnected=off
  wires:
  Demux3/14 -> Bus Creator3/14  "Vhcl Wheel RR Trq_WhlBearing"
  Demux3/13 -> Bus Creator3/13  "Vhcl Wheel RR Trq_T2W"
  Demux3/12 -> Bus Creator3/12  "Vhcl Wheel RR SideSlip"
  Demux3/11 -> Bus Creator3/11  "Vhcl Wheel RR LongSlip"
  Demux3/10 -> Bus Creator3/10  "Vhcl Wheel RR vBelt"
  Demux3/9 -> Bus Creator3/9  "Vhcl Wheel RR Fz"
  Demux3/8 -> Bus Creator3/8  "Vhcl Wheel RR Fy"
  Demux3/7 -> Bus Creator3/7  "Vhcl Wheel RR Fx"
  Demux3/6 -> Bus Creator3/6  "Vhcl Wheel RR r_zxy z"
  Demux3/5 -> Bus Creator3/5  "Vhcl Wheel RR r_zxy y"
  Demux3/4 -> Bus Creator3/4  "Vhcl Wheel RR r_zxy x"
  Demux3/3 -> Bus Creator3/3  "Vhcl Wheel RR t z"
  Demux3/2 -> Bus Creator3/2  "Vhcl Wheel RR t y"
  In1/1 -> Demux3/1
  Bus Creator3/1 -> Out1/1
  Demux3/1 -> Bus Creator3/1  "Vhcl Wheel RR t x"

== system generic_src/CarMaker/IPG Vehicle/PowerTrain/MCU Example/CreateBus MCU ISGOut ==
  In : Inport
  BusCreator : BusCreator  Inputs=8
  Demux : Demux  Outputs=8
      settings: DisplayOption=none
  Out : Outport  VectorParamsAs1DForOutWhenUnconnected=off
  wires:
  In/1 -> Demux/1
  Demux/5 -> BusCreator/5  "MCU ISGOut Voltage_q"
  Demux/2 -> BusCreator/2  "MCU ISGOut TrqMot_max"
  Demux/1 -> BusCreator/1  "MCU ISGOut Load"
  Demux/7 -> BusCreator/7  "MCU ISGOut Voltage_v"
  Demux/8 -> BusCreator/8  "MCU ISGOut Voltage_w"
  Demux/6 -> BusCreator/6  "MCU ISGOut Voltage_u"
  Demux/4 -> BusCreator/4  "MCU ISGOut Voltage_d"
  Demux/3 -> BusCreator/3  "MCU ISGOut TrqGen_max"
  BusCreator/1 -> Out/1

== system generic_src/CarMaker/IPG Vehicle/PowerTrain/MCU Example/CreateBus MCU MotorOut0 ==
  In : Inport
  BusCreator1 : BusCreator  Inputs=8
  Demux1 : Demux  Outputs=8
      settings: DisplayOption=none
  Out : Outport  VectorParamsAs1DForOutWhenUnconnected=off
  wires:
  BusCreator1/1 -> Out/1
  Demux1/3 -> BusCreator1/3  "MCU MotorOut0 TrqGen_max"
  Demux1/2 -> BusCreator1/2  "MCU MotorOut0 TrqMot_max"
  Demux1/7 -> BusCreator1/7  "MCU MotorOut0 Voltage_v"
  Demux1/1 -> BusCreator1/1  "MCU MotorOut0 Load"
  In/1 -> Demux1/1
  Demux1/4 -> BusCreator1/4  "MCU MotorOut0 Voltage_d"
  Demux1/5 -> BusCreator1/5  "MCU MotorOut0 Voltage_q"
  Demux1/8 -> BusCreator1/8  "MCU MotorOut0 Voltage_w"
  Demux1/6 -> BusCreator1/6  "MCU MotorOut0 Voltage_u"

== system generic_src/CarMaker/IPG Vehicle/PowerTrain/MCU Example/CreateBus MCU MotorOut1 ==
  In : Inport
  BusCreator1 : BusCreator  Inputs=8
  Demux1 : Demux  Outputs=8
      settings: DisplayOption=none
  Out : Outport  VectorParamsAs1DForOutWhenUnconnected=off
  wires:
  Demux1/6 -> BusCreator1/6  "MCU MotorOut1 Voltage_u"
  Demux1/7 -> BusCreator1/7  "MCU MotorOut1 Voltage_v"
  BusCreator1/1 -> Out/1
  Demux1/3 -> BusCreator1/3  "MCU MotorOut1 TrqGen_max"
  Demux1/1 -> BusCreator1/1  "MCU MotorOut1 Load"
  In/1 -> Demux1/1
  Demux1/8 -> BusCreator1/8  "MCU MotorOut1 Voltage_w"
  Demux1/2 -> BusCreator1/2  "MCU MotorOut1 TrqMot_max"
  Demux1/4 -> BusCreator1/4  "MCU MotorOut1 Voltage_d"
  Demux1/5 -> BusCreator1/5  "MCU MotorOut1 Voltage_q"

== system generic_src/CarMaker/IPG Vehicle/PowerTrain/MCU Example/CreateBus MCU MotorOut2 ==
  In : Inport
  BusCreator1 : BusCreator  Inputs=8
  Demux1 : Demux  Outputs=8
      settings: DisplayOption=none
  Out : Outport  VectorParamsAs1DForOutWhenUnconnected=off
  wires:
  Demux1/1 -> BusCreator1/1  "MCU MotorOut2 Load"
  Demux1/3 -> BusCreator1/3  "MCU MotorOut2 TrqGen_max"
  BusCreator1/1 -> Out/1
  Demux1/8 -> BusCreator1/8  "MCU MotorOut2 Voltage_w"
  Demux1/4 -> BusCreator1/4  "MCU MotorOut2 Voltage_d"
  In/1 -> Demux1/1
  Demux1/6 -> BusCreator1/6  "MCU MotorOut2 Voltage_u"
  Demux1/2 -> BusCreator1/2  "MCU MotorOut2 TrqMot_max"
  Demux1/5 -> BusCreator1/5  "MCU MotorOut2 Voltage_q"
  Demux1/7 -> BusCreator1/7  "MCU MotorOut2 Voltage_v"

== system generic_src/CarMaker/IPG Vehicle/PowerTrain/MCU Example/CreateBus MCU MotorOut3 ==
  In : Inport
  BusCreator1 : BusCreator  Inputs=8
  Demux1 : Demux  Outputs=8
      settings: DisplayOption=none
  Out : Outport  VectorParamsAs1DForOutWhenUnconnected=off
  wires:
  Demux1/7 -> BusCreator1/7  "MCU MotorOut3 Voltage_v"
  Demux1/3 -> BusCreator1/3  "MCU MotorOut3 TrqGen_max"
  Demux1/1 -> BusCreator1/1  "MCU MotorOut3 Load"
  Demux1/5 -> BusCreator1/5  "MCU MotorOut3 Voltage_q"
  Demux1/8 -> BusCreator1/8  "MCU MotorOut3 Voltage_w"
  Demux1/4 -> BusCreator1/4  "MCU MotorOut3 Voltage_d"
  Demux1/6 -> BusCreator1/6  "MCU MotorOut3 Voltage_u"
  BusCreator1/1 -> Out/1
  In/1 -> Demux1/1
  Demux1/2 -> BusCreator1/2  "MCU MotorOut3 TrqMot_max"

== system generic_src/CarMaker/IPG Vehicle/PowerTrain/MCU Example/CreateBus MCU Status ==
  In : Inport
  BusCreator : BusCreator  Inputs=1
  Demux : Demux  Outputs=1
      settings: DisplayOption=none
  Out : Outport  VectorParamsAs1DForOutWhenUnconnected=off
  wires:
  Demux/1 -> BusCreator/1  "MCU_Out Status"
  In/1 -> Demux/1
  BusCreator/1 -> Out/1

== system generic_src/CarMaker/IPG Vehicle/PowerTrain/MCU Example/MyMotorCU ==
  Ignition : Inport
  rotv : Inport  Port=2
  Trq_trg : Inport  Port=3
  Load : Inport  Port=4
  rotv_trg : Inport  Port=5
  CfgIF : Inport  Port=6
  Bus Creator : BusCreator  Inputs=3
  Bus Selector : BusSelector  OutputSignals=MCU_Cfg ISG Ratio,TrqMot_max,TrqGen_max,MCU_Cfg ISG rotv_Mot_max,MCU_Cfg ISG rotv_Gen_max
  Bus Selector1 : BusSelector  OutputSignals=Load,TrqMot_max,TrqGen_max
  Enabled Subsystem : Subsystem  TreatAsAtomicUnit=on
  Logical Operator : Logic  Operator=NOT  AllPortsSameDT=off  OutDataTypeStr=boolean
  Merge : Merge
  ReturnZero : Subsystem  TreatAsAtomicUnit=on
  Load out : Outport  VectorParamsAs1DForOutWhenUnconnected=off
  TrqMot_max : Outport  Port=2  VectorParamsAs1DForOutWhenUnconnected=off
  TrqGen_max : Outport  Port=3  VectorParamsAs1DForOutWhenUnconnected=off
  wires:
  Bus Selector1/1 -> Load out/1  "<Load>"
  Bus Selector1/2 -> TrqMot_max/1  "<TrqMot_max>"
  Bus Selector1/3 -> TrqGen_max/1  "<TrqGen_max>"
  Merge/1 -> Bus Selector1/1
  Bus Creator/1 -> Merge/2
  ReturnZero/1(ReturnZero) -> Merge/1
  Enabled Subsystem/3(TrqGen_max) -> Bus Creator/3  "TrqGen_max"
  Enabled Subsystem/2(TrqMot_max) -> Bus Creator/2  "TrqMot_max"
  Enabled Subsystem/1(Load out) -> Bus Creator/1  "Load"
  rotv_trg/1 -> Enabled Subsystem/4(rotv_trg)
  Load/1 -> Enabled Subsystem/3(Load)
  Trq_trg/1 -> Enabled Subsystem/2(Trq_trg)
  Bus Selector/5 -> Enabled Subsystem/9(rotv_Gen_max)  "<MCU_Cfg ISG rotv_Gen_max>"
  Bus Selector/4 -> Enabled Subsystem/8(rotv_Mot_max)  "<MCU_Cfg ISG rotv_Mot_max>"
  Bus Selector/3 -> Enabled Subsystem/7(TrqGen_max table)  "<TrqGen_max>"
  Bus Selector/2 -> Enabled Subsystem/6(TrqMot_max table)  "<TrqMot_max >"
  Bus Selector/1 -> Enabled Subsystem/5(Ratio)  "<MCU_Cfg ISG Ratio>"
  CfgIF/1 -> Bus Selector/1
  rotv/1 -> Enabled Subsystem/1(rotv)
  Logical Operator/1 -> ReturnZero/Enable
  Ignition/1 -> Logical Operator/1, Enabled Subsystem/Enable

== system generic_src/CarMaker/IPG Vehicle/PowerTrain/MCU Example/PTMotorCU_In ==
  Sync_In : Inport
  CreateBus MCU ISGIn : Subsystem
  CreateBus MCU ISGOut : Subsystem
  CreateBus MCU Ignition : Subsystem
  CreateBus MCU MotorIn0 : Subsystem
  CreateBus MCU MotorIn1 : Subsystem
  CreateBus MCU MotorIn2 : Subsystem
  CreateBus MCU MotorIn3 : Subsystem
  CreateBus MCU MotorOut0 : Subsystem
  CreateBus MCU MotorOut1 : Subsystem
  CreateBus MCU MotorOut2 : Subsystem
  CreateBus MCU MotorOut3 : Subsystem
  CreateBus MCU_Cfg ISG : Subsystem
  CreateBus MCU_Cfg Misc : Subsystem
  CreateBus MCU_Cfg Motor0 : Subsystem
  CreateBus MCU_Cfg Motor1 : Subsystem
  CreateBus MCU_Cfg Motor2 : Subsystem
  CreateBus MCU_Cfg Motor3 : Subsystem
  CreateBus PTMotorCU_In : BusCreator  Inputs=17
  S-Function : S-Function  FunctionName=cm_ptmotorcu_in  SFunctionDeploymentMode=off  EnableBusSupport=off
  PTMotorCU_In : Outport  VectorParamsAs1DForOutWhenUnconnected=off
  wires:
  S-Function/17 -> CreateBus MCU MotorOut3/1(In)
  S-Function/16 -> CreateBus MCU MotorOut2/1(In)
  S-Function/15 -> CreateBus MCU MotorOut1/1(In)
  S-Function/12 -> CreateBus MCU MotorIn2/1(In)
  S-Function/10 -> CreateBus MCU MotorIn0/1(In)
  CreateBus MCU MotorIn0/1(Out) -> CreateBus PTMotorCU_In/10  "MCU MotorIn0"
  CreateBus MCU ISGIn/1(Out) -> CreateBus PTMotorCU_In/8  "MCU ISGIn"
  CreateBus MCU MotorIn2/1(Out) -> CreateBus PTMotorCU_In/12  "MCU MotorIn2"
  S-Function/8 -> CreateBus MCU ISGIn/1(In)
  CreateBus MCU_Cfg ISG/1(Out) -> CreateBus PTMotorCU_In/2  "MCU_Cfg ISG"
  CreateBus MCU MotorIn3/1(Out) -> CreateBus PTMotorCU_In/13  "MCU MotorIn3"
  CreateBus MCU MotorIn1/1(Out) -> CreateBus PTMotorCU_In/11  "MCU MotorIn1"
  S-Function/14 -> CreateBus MCU MotorOut0/1(In)
  S-Function/13 -> CreateBus MCU MotorIn3/1(In)
  S-Function/11 -> CreateBus MCU MotorIn1/1(In)
  CreateBus MCU ISGOut/1(Out) -> CreateBus PTMotorCU_In/9  "MCU ISGOut"
  CreateBus MCU_Cfg Misc/1(Out) -> CreateBus PTMotorCU_In/1  "MCU_Cfg Misc"
  CreateBus MCU Ignition/1(Out) -> CreateBus PTMotorCU_In/7  "MCU Ignition"
  S-Function/3 -> CreateBus MCU_Cfg Motor0/1(In)
  Sync_In/1 -> S-Function/1
  CreateBus MCU MotorOut2/1(Out) -> CreateBus PTMotorCU_In/16  "MCU MotorOut2"
  CreateBus MCU MotorOut0/1(Out) -> CreateBus PTMotorCU_In/14  "MCU MotorOut0"
  CreateBus MCU MotorOut1/1(Out) -> CreateBus PTMotorCU_In/15  "MCU MotorOut1"
  CreateBus MCU_Cfg Motor2/1(Out) -> CreateBus PTMotorCU_In/5  "MCU_Cfg Motor2"
  S-Function/2 -> CreateBus MCU_Cfg ISG/1(In)
  CreateBus MCU_Cfg Motor3/1(Out) -> CreateBus PTMotorCU_In/6  "MCU_Cfg Motor3"
  S-Function/5 -> CreateBus MCU_Cfg Motor2/1(In)
  CreateBus MCU_Cfg Motor1/1(Out) -> CreateBus PTMotorCU_In/4  "MCU_Cfg Motor1"
  S-Function/1 -> CreateBus MCU_Cfg Misc/1(In)
  S-Function/4 -> CreateBus MCU_Cfg Motor1/1(In)
  CreateBus MCU_Cfg Motor0/1(Out) -> CreateBus PTMotorCU_In/3  "MCU_Cfg Motor0"
  CreateBus PTMotorCU_In/1 -> PTMotorCU_In/1
  CreateBus MCU MotorOut3/1(Out) -> CreateBus PTMotorCU_In/17  "MCU MotorOut3"
  S-Function/9 -> CreateBus MCU ISGOut/1(In)
  S-Function/6 -> CreateBus MCU_Cfg Motor3/1(In)
  S-Function/7 -> CreateBus MCU Ignition/1(In)

== system generic_src/CarMaker/IPG Vehicle/PowerTrain/MCU Example/PTMotorCU_Out ==
  MCU Status : Inport
  MCU ISGOut : Inport  Port=2
  MCU MotorOut0 : Inport  Port=3
  MCU MotorOut1 : Inport  Port=4
  MCU MotorOut2 : Inport  Port=5
  MCU MotorOut3 : Inport  Port=6
  S-Function : S-Function  FunctionName=cm_ptmotorcu_out  SFunctionDeploymentMode=off  EnableBusSupport=off
  wires:
  MCU MotorOut3/1 -> S-Function/6
  MCU MotorOut1/1 -> S-Function/4
  MCU MotorOut0/1 -> S-Function/3
  MCU MotorOut2/1 -> S-Function/5
  MCU Status/1 -> S-Function/1
  MCU ISGOut/1 -> S-Function/2

== system generic_src/CarMaker/IPG Vehicle/PowerTrain/PTControl Example/CreateBus PTC BatteryHVOut ==
  In : Inport
  BusCreator : BusCreator  Inputs=2
  Demux : Demux  Outputs=2
      settings: DisplayOption=none
  Out : Outport  VectorParamsAs1DForOutWhenUnconnected=off
  wires:
  Demux/2 -> BusCreator/2  "PTC BattHVOut MassFlowCool_trg"
  Demux/1 -> BusCreator/1  "PTC BattHVOut Temp_trg"
  In/1 -> Demux/1
  BusCreator/1 -> Out/1

== system generic_src/CarMaker/IPG Vehicle/PowerTrain/PTControl Example/CreateBus PTC BatteryLVOut ==
  In : Inport
  BusCreator : BusCreator  Inputs=2
  Demux : Demux  Outputs=2
      settings: DisplayOption=none
  Out : Outport  VectorParamsAs1DForOutWhenUnconnected=off
  wires:
  Demux/2 -> BusCreator/2  "PTC BattLVOut MassFlowCool_trg"
  In/1 -> Demux/1
  Demux/1 -> BusCreator/1  "PTC BattLVOut Temp_trg"
  BusCreator/1 -> Out/1

== system generic_src/CarMaker/IPG Vehicle/PowerTrain/PTControl Example/CreateBus PTC EngineOut ==
  In : Inport
  BusCreator : BusCreator  Inputs=5
  Demux : Demux  Outputs=5
      settings: DisplayOption=none
  Out : Outport  VectorParamsAs1DForOutWhenUnconnected=off
  wires:
  Demux/5 -> BusCreator/5  "PTC EngineOut rotv_trg"
  Demux/4 -> BusCreator/4  "PTC EngineOut Trq_trg"
  Demux/3 -> BusCreator/3  "PTC EngineOut Load"
  Demux/2 -> BusCreator/2  "PTC EngineOut FuelCutOff"
  Demux/1 -> BusCreator/1  "PTC EngineOut set_ISC"
  BusCreator/1 -> Out/1
  In/1 -> Demux/1

== system generic_src/CarMaker/IPG Vehicle/PowerTrain/PTControl Example/CreateBus PTC ISGOut ==
  In : Inport
  BusCreator : BusCreator  Inputs=3
  Demux : Demux  Outputs=3
      settings: DisplayOption=none
  Out : Outport  VectorParamsAs1DForOutWhenUnconnected=off
  wires:
  Demux/3 -> BusCreator/3  "PTC ISGOut rotv_trg"
  Demux/2 -> BusCreator/2  "PTC ISGOut Trq_trg"
  Demux/1 -> BusCreator/1  "PTC ISGOut Load"
  BusCreator/1 -> Out/1
  In/1 -> Demux/1

== system generic_src/CarMaker/IPG Vehicle/PowerTrain/PTControl Example/CreateBus PTC MiscOut ==
  In : Inport
  BusCreator : BusCreator  Inputs=4
  Demux : Demux
      settings: DisplayOption=none
  Out : Outport  VectorParamsAs1DForOutWhenUnconnected=off
  wires:
  Demux/4 -> BusCreator/4  "PTC_Out Ignition"
  Demux/3 -> BusCreator/3  "PTC_Out StrategyMode"
  Demux/2 -> BusCreator/2  "PTC_Out OperationError"
  Demux/1 -> BusCreator/1  "PTC_Out OperationState"
  BusCreator/1 -> Out/1
  In/1 -> Demux/1

== system generic_src/CarMaker/IPG Vehicle/PowerTrain/PTControl Example/CreateBus PTC PwrSupplyOut ==
  In : Inport
  BusCreator : BusCreator  Inputs=1
  Demux : Demux  Outputs=1
      settings: DisplayOption=none
  Out : Outport  VectorParamsAs1DForOutWhenUnconnected=off
  wires:
  Demux/1 -> BusCreator/1  "PTC PwrSupplyOut Pwr_HV1toLV_trg"
  BusCreator/1 -> Out/1
  In/1 -> Demux/1

== system generic_src/CarMaker/IPG Vehicle/PowerTrain/PTControl Example/CreateBus PTC WheelOut ==
  In : Inport
  BusCreator : BusCreator  Inputs=8
  Demux : Demux  Outputs=8
      settings: DisplayOption=none
  Out : Outport  VectorParamsAs1DForOutWhenUnconnected=off
  wires:
  Demux/8 -> BusCreator/8  "PTC WheelOut_RR Trq_BrakeReg_max"
  Demux/7 -> BusCreator/7  "PTC WheelOut_RR Trq_BrakeReg"
  Demux/6 -> BusCreator/6  "PTC WheelOut_RL Trq_BrakeReg_max"
  Demux/5 -> BusCreator/5  "PTC WheelOut_RL Trq_BrakeReg"
  Demux/4 -> BusCreator/4  "PTC WheelOut_FR Trq_BrakeReg_max"
  Demux/3 -> BusCreator/3  "PTC WheelOut_FR Trq_BrakeReg"
  Demux/2 -> BusCreator/2  "PTC WheelOut_FL Trq_BrakeReg_max"
  Demux/1 -> BusCreator/1  "PTC WheelOut_FL Trq_BrakeReg"
  BusCreator/1 -> Out/1
  In/1 -> Demux/1

== system generic_src/CarMaker/IPG Vehicle/PowerTrain/PTControl Example/PTC ClutchOut ==
  ClutchOut Pos : Inport
  Bus Assignment : BusAssignment  AssignedSignals=PTC ClutchOut0 Pos
  BusCreator : BusCreator  Inputs=12
  CreateBus PTC ClutchOut0 : Subsystem
  CreateBus PTC ClutchOut1 : Subsystem
  CreateBus PTC ClutchOut10 : Subsystem
  CreateBus PTC ClutchOut11 : Subsystem
  CreateBus PTC ClutchOut2 : Subsystem
  CreateBus PTC ClutchOut3 : Subsystem
  CreateBus PTC ClutchOut4 : Subsystem
  CreateBus PTC ClutchOut5 : Subsystem
  CreateBus PTC ClutchOut6 : Subsystem
  CreateBus PTC ClutchOut7 : Subsystem
  CreateBus PTC ClutchOut8 : Subsystem
  CreateBus PTC ClutchOut9 : Subsystem
  Ground PTC GearBoxOut{1..12} (12 alike) : Ground
  PTC ClutchOut : Outport
  wires:
  ClutchOut Pos/1 -> Bus Assignment/2
  CreateBus PTC ClutchOut0/1(Out) -> Bus Assignment/1
  Ground PTC GearBoxOut4/1 -> CreateBus PTC ClutchOut0/1(In)
  Ground PTC GearBoxOut3/1 -> CreateBus PTC ClutchOut1/1(In)
  Ground PTC GearBoxOut2/1 -> CreateBus PTC ClutchOut2/1(In)
  Ground PTC GearBoxOut1/1 -> CreateBus PTC ClutchOut3/1(In)
  Ground PTC GearBoxOut5/1 -> CreateBus PTC ClutchOut4/1(In)
  Ground PTC GearBoxOut6/1 -> CreateBus PTC ClutchOut5/1(In)
  Ground PTC GearBoxOut7/1 -> CreateBus PTC ClutchOut6/1(In)
  Ground PTC GearBoxOut8/1 -> CreateBus PTC ClutchOut7/1(In)
  Ground PTC GearBoxOut9/1 -> CreateBus PTC ClutchOut8/1(In)
  Ground PTC GearBoxOut10/1 -> CreateBus PTC ClutchOut9/1(In)
  Ground PTC GearBoxOut11/1 -> CreateBus PTC ClutchOut10/1(In)
  Ground PTC GearBoxOut12/1 -> CreateBus PTC ClutchOut11/1(In)
  Bus Assignment/1 -> BusCreator/1  "PTC ClutchOut0"
  CreateBus PTC ClutchOut1/1(Out) -> BusCreator/2  "PTC ClutchOut1"
  CreateBus PTC ClutchOut2/1(Out) -> BusCreator/3  "PTC ClutchOut2"
  CreateBus PTC ClutchOut3/1(Out) -> BusCreator/4  "PTC ClutchOut3"
  CreateBus PTC ClutchOut4/1(Out) -> BusCreator/5  "PTC ClutchOut4"
  CreateBus PTC ClutchOut5/1(Out) -> BusCreator/6  "PTC ClutchOut5"
  CreateBus PTC ClutchOut6/1(Out) -> BusCreator/7  "PTC ClutchOut6"
  CreateBus PTC ClutchOut7/1(Out) -> BusCreator/8  "PTC ClutchOut7"
  CreateBus PTC ClutchOut8/1(Out) -> BusCreator/9  "PTC ClutchOut8"
  CreateBus PTC ClutchOut9/1(Out) -> BusCreator/10  "PTC ClutchOut9"
  CreateBus PTC ClutchOut10/1(Out) -> BusCreator/11  "PTC ClutchOut10"
  CreateBus PTC ClutchOut11/1(Out) -> BusCreator/12  "PTC ClutchOut11"
  BusCreator/1 -> PTC ClutchOut/1  "PTC ClutchOut"

== system generic_src/CarMaker/IPG Vehicle/PowerTrain/PTControl Example/PTC GearBoxOut ==
  GearBoxOut GearNoTrg : Inport
  Bus Assignment1 : BusAssignment  AssignedSignals=PTC GearboxOut0 GearNoTrg
  BusCreator : BusCreator  Inputs=12
  CreateBus PTC GearboxOut0 : Subsystem
  CreateBus PTC GearboxOut1 : Subsystem
  CreateBus PTC GearboxOut10 : Subsystem
  CreateBus PTC GearboxOut11 : Subsystem
  CreateBus PTC GearboxOut2 : Subsystem
  CreateBus PTC GearboxOut3 : Subsystem
  CreateBus PTC GearboxOut4 : Subsystem
  CreateBus PTC GearboxOut5 : Subsystem
  CreateBus PTC GearboxOut6 : Subsystem
  CreateBus PTC GearboxOut7 : Subsystem
  CreateBus PTC GearboxOut8 : Subsystem
  CreateBus PTC GearboxOut9 : Subsystem
  Ground PTC GearboxOut{0..11} (12 alike) : Ground
  PTC GearboxOut : Outport
  wires:
  GearBoxOut GearNoTrg/1 -> Bus Assignment1/2
  Ground PTC GearboxOut0/1 -> CreateBus PTC GearboxOut0/1(In)
  CreateBus PTC GearboxOut0/1(Out) -> Bus Assignment1/1
  Ground PTC GearboxOut3/1 -> CreateBus PTC GearboxOut3/1(In)
  Ground PTC GearboxOut2/1 -> CreateBus PTC GearboxOut2/1(In)
  Ground PTC GearboxOut1/1 -> CreateBus PTC GearboxOut1/1(In)
  Ground PTC GearboxOut4/1 -> CreateBus PTC GearboxOut4/1(In)
  Ground PTC GearboxOut5/1 -> CreateBus PTC GearboxOut5/1(In)
  Ground PTC GearboxOut6/1 -> CreateBus PTC GearboxOut6/1(In)
  Ground PTC GearboxOut7/1 -> CreateBus PTC GearboxOut7/1(In)
  Ground PTC GearboxOut8/1 -> CreateBus PTC GearboxOut8/1(In)
  Ground PTC GearboxOut9/1 -> CreateBus PTC GearboxOut9/1(In)
  Ground PTC GearboxOut10/1 -> CreateBus PTC GearboxOut10/1(In)
  Ground PTC GearboxOut11/1 -> CreateBus PTC GearboxOut11/1(In)
  Bus Assignment1/1 -> BusCreator/1  "PTC GearBoxOut0"
  CreateBus PTC GearboxOut1/1(Out) -> BusCreator/2  "PTC GearBoxOut1"
  CreateBus PTC GearboxOut2/1(Out) -> BusCreator/3  "PTC GearBoxOut2"
  CreateBus PTC GearboxOut3/1(Out) -> BusCreator/4  "PTC GearBoxOut3"
  CreateBus PTC GearboxOut4/1(Out) -> BusCreator/5  "PTC GearBoxOut4"
  CreateBus PTC GearboxOut5/1(Out) -> BusCreator/6  "PTC GearBoxOut5"
  CreateBus PTC GearboxOut6/1(Out) -> BusCreator/7  "PTC GearBoxOut6"
  CreateBus PTC GearboxOut7/1(Out) -> BusCreator/8  "PTC GearBoxOut7"
  CreateBus PTC GearboxOut8/1(Out) -> BusCreator/9  "PTC GearBoxOut8"
  CreateBus PTC GearboxOut9/1(Out) -> BusCreator/10  "PTC GearBoxOut9"
  CreateBus PTC GearboxOut10/1(Out) -> BusCreator/11  "PTC GearBoxOut10"
  CreateBus PTC GearboxOut11/1(Out) -> BusCreator/12  "PTC GearBoxOut11"
  BusCreator/1 -> PTC GearboxOut/1  "PTC GearboxOut"
